simulink library "mjLib"  (R2025b)
settings: Solver=VariableStepAuto  StartTime=0.0  StopTime=10.0  RelTol=1e-3
settings Model: Creator=vmano  LastModifiedBy=Junch
settings OptimizationCC: ReuseModelBlockBuffer=off
settings DebuggingCC: UnconnectedInputMsg=warning  UnconnectedOutputMsg=warning  UnconnectedLineMsg=warning
settings ModelReferenceCC: EnableRefExpFcnMdlSchedulingChecks=on
settings RTWCC: GPUComputeCapability=3.5  DLArmComputeVersion=19.05

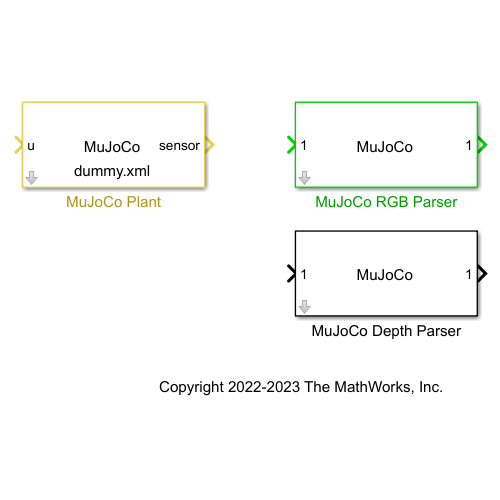
[thumbnail: Simulink's stored preview of the top-level diagram]
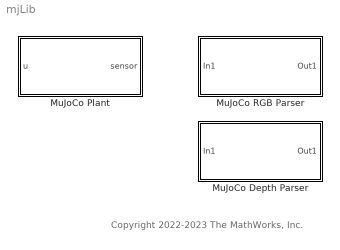
== system mjLib ==
  note: Copyright 2022-2023 The MathWorks, Inc.
  MuJoCo Depth Parser : Subsystem  mask{inputBusType=mj_bus_rgb_6338524502533525485, selectedCamera=camera, imageRows=480, imageCols=640, startingIndex=1, endingIndex=307200}
      mask prompts: inputBusType "Input Type"; selectedCamera "Select Camera"
      mask TypeOptions inputBusType: mj_bus_rgb_6338524502533525485
      mask Callback inputBusType:
      | inputBusType = get_param(gcb, 'inputBusType');
      | 
      | inputStruct = Simulink.Bus.createMATLABStruct(inputBusType);
      | 
      | mo = Simulink.Mask.get(gcb);
      | mo.Parameters(2).TypeOptions = fieldnames(inputStruct);
      mask TypeOptions selectedCamera: camera
      mask Callback selectedCamera:
      | inputBusType = get_param(gcb, 'inputBusType');
      | selectedCamera = get_param(gcb, 'selectedCamera');
      | 
      | inputStruct = Simulink.Bus.createMATLABStruct(inputBusType);
      | imageSize = size(inputStruct.(selectedCamera));
      | 
      | imageRows = imageSize(1);
      | imageCols = imageSize(2);
      | 
      | set_param(gcb, 'imageRows', num2str(imageRows));
      | set_param(gcb, 'imageCols', num2str(imageCols));
      | 
      | fields = fieldnames(inputStruct);
      | [~, camIndex] = ismember(selectedCamera, fields);
      | 
      | startingIndex = 1;
      | for i=1:(camIndex-1)
      |     imageSize = size(inputStruct.(fields{i}));
      |     startingIndex = startingIndex + imageSize(1)*imageSize(2);
      | end
      | endingIndex = startingIndex+imageSize(1) * imageSize(2) - 1;
      | 
      | set_param(gcb, 'startingIndex', num2str(startingIndex));
      | set_param(gcb, 'endingIndex', num2str(endingIndex));
      mask DialogControl Control2 Prompt: Refresh
      mask DialogControl Control2 Callback:
      | mo = Simulink.Mask.get(gcb);
      | mo.Parameters(1).TypeOptions = evalin('base', "who('mj_bus_rgb*')");
      mask Display:
      | color('black')
      | text(0.5, 0.5, 'MuJoCo', 'horizontalAlignment', 'center')
  MuJoCo Plant : Subsystem  mask(MuJoCo Plant){controlBus=[], sensorBus=mj_bus_sensor_7979902499018342666, controlLength=[], sensorLength=[], rgbLength=[], depthLength=[], sampleTime=0.005, xmlFileRel=dummy.xml, xmlFile=D:\robotics\mujoco_blocks\dummy.xml, renderingType=Global, vsync=off, visualFPS=60, zoomLevel=1, windowWidth=800, windowHeight=800, showSiteTrajectory=off, trajectorySiteName=, znear=0.059256, zfar=296.2816, cameraOutputEnabled=off, cameraSampleTime=0.020, rgbOutOption=on, depthOutOption=off, controlInterfaceType=Vector}
      mask prompts: renderingType "Type"; visualFPS "FPS"; zoomLevel "Zoom"; windowWidth "Window width (px)"; windowHeight "Window height (px)"; showSiteTrajectory "Show Site Trajectory"; trajectorySiteName "Site Name"; cameraOutputEnabled "Camera Output"; cameraSampleTime "Sample Time"; rgbOutOption "RGB Output"; depthOutOption "Depth Output"; controlInterfaceType "Interface"
      mask help:
      | This block provides an interface to MuJoCo™ physics engine.
      | It sets control inputs, steps the engine and outputs sensor/camera.
      |
      | Inputs, sensors, cameras and sample time information is obtained from the model XML.
      |
      | Control inputs are provided either as a non-virtual bus or vector.
      | Sensors are output as a non-virtual bus.
      | Camera data is output as a vector which can be decoded using MuJoCo RGB/Depth Parser blocks.
      mask init:
      | [controlBus, sensorBus, rgbBus, depthBus, dataLengths] = mj_initbus(xmlFile, cameraOutputEnabled);
      |     controlLength = double(dataLengths(1));
      |     sensorLength = double(dataLengths(2));
      |     rgbLength = double(dataLengths(3));
      |     depthLength = double(dataLengths(4)) * double(depthOutOption);
      |     mj_maskinit;
      mask Callback xmlFileRel:
      | relpath = get_param(gcb, 'xmlFileRel');
      | 
      | abspath = which(relpath);
      | if isempty(abspath)
      |     abspath = relpath;
      | end
      | set_param(gcb, 'xmlFile', abspath);
      mask TypeOptions renderingType: Local | Global | None
      mask TypeOptions controlInterfaceType: Bus | Vector
      mask DialogControl Container3 Prompt: Model Info
      mask DialogControl controlBusText Prompt: Control Vector Type: [armMotor]
      mask DialogControl sensorBusText Prompt: Sensor Bus Type: mj_bus_sensor_15738467249377022003
      mask DialogControl rgbBusText Prompt: RGB Bus Type: NA
      mask DialogControl depthBusText Prompt: Depth Bus Type: NA
      mask DialogControl sampleTimeText Prompt: Sample Time: 0.005
      mask DialogControl Container10 Prompt: Model
      mask DialogControl getFileButton Prompt: Browse
      mask DialogControl getFileButton Callback:
      | oldPath = get_param(gcb, 'xmlFile');
      | [file, path] = uigetfile({'*.xml;*.urdf'}, 'File Selector', oldPath);
      | if file~=0
      |     xml = fullfile(path, file);
      |     set_param(gcb, 'xmlFileRel', xml);
      | end
      mask DialogControl testStandaloneButton Prompt: Test
      mask DialogControl testStandaloneButton Callback: disp('Not implemented yet. Call simulate.exe inside 3p/mujoco folder')
      mask DialogControl Container12 Prompt: Rendering
      mask DialogControl Control11 Prompt: Rendering thread is common to all MuJoCo blocks and is used for rendering visualizer window along with all cameras
      mask DialogControl Container9 Prompt: Visualizer
      mask DialogControl Control10 Prompt: Visualizer renders frames at specified FPS. Display buffer swap timing is controlled separately via vsync option.
      mask DialogControl renderingType Tooltip: Local rendering creates a unique window for each MuJoCo block. Global tries to merge different block visuals into one window. None disables visualization
      mask DialogControl Container11 Prompt: Options
      mask DialogControl vsync Tooltip: Vsync blocks rendering thread until the monitor is ready to show the next frame. This prevents screen tearing effect. Vsync can slow down everything including physics loop.
      mask DialogControl visualFPS Tooltip: If Vsync is disabled, specify the FPS to show visuals at.
      mask DialogControl windowWidth Tooltip: Initial width of the visualization window. For Global rendering, the block that creates the shared window sets its size.
      mask DialogControl windowHeight Tooltip: Initial height of the visualization window. For Global rendering, the block that creates the shared window sets its size.
      mask DialogControl showSiteTrajectory Tooltip: Draw the world-space path of the selected site in the Local or Global window.
      mask DialogControl trajectorySiteName Tooltip: Exact name of a site in the loaded MJCF model. Required when Show Site Trajectory is selected.
      mask DialogControl Container13 Prompt: Camera
      mask DialogControl Control9 Prompt: Camera rendering runs in lockstep with physics engine.
      mask DialogControl cameraOutputEnabled Tooltip: Enable offscreen camera rendering and RGB/depth output ports.
      mask DialogControl depthOutOption Tooltip: Disable depth buffer processing to improve simulation speed.
      mask DialogControl Container7 Prompt: Control Inputs
      mask Display:
      | color('black')
      | text(0.5, 0.5, 'MuJoCo', 'horizontalAlignment', 'center')
      | [~, nameText, ext] = fileparts(get_param(gcb, 'xmlFile'));
      | text(0.5, 0.2, [nameText, ext], 'horizontalAlignment', 'center')
  MuJoCo RGB Parser : Subsystem  mask{inputBusType=mj_bus_rgb_6338524502533525485, selectedCamera=camera, imageRows=480, imageCols=640, startingIndex=1, endingIndex=921600}
      mask prompts: inputBusType "Input Type"; selectedCamera "Select Camera"
      mask TypeOptions inputBusType: mj_bus_rgb_4478678753310125630 | mj_bus_rgb_4479672711821839149
      mask Callback inputBusType:
      | inputBusType = get_param(gcb, 'inputBusType');
      | 
      | inputStruct = Simulink.Bus.createMATLABStruct(inputBusType);
      | 
      | mo = Simulink.Mask.get(gcb);
      | mo.Parameters(2).TypeOptions = fieldnames(inputStruct);
      mask TypeOptions selectedCamera: camera
      mask Callback selectedCamera:
      | inputBusType = get_param(gcb, 'inputBusType');
      | selectedCamera = get_param(gcb, 'selectedCamera');
      | 
      | inputStruct = Simulink.Bus.createMATLABStruct(inputBusType);
      | imageSize = size(inputStruct.(selectedCamera));
      | 
      | imageRows = imageSize(1);
      | imageCols = imageSize(2);
      | 
      | set_param(gcb, 'imageRows', num2str(imageRows));
      | set_param(gcb, 'imageCols', num2str(imageCols));
      | 
      | fields = fieldnames(inputStruct);
      | [~, camIndex] = ismember(selectedCamera, fields);
      | 
      | startingIndex = 1;
      | for i=1:(camIndex-1)
      |     imageSize = size(inputStruct.(fields{i}));
      |     startingIndex = startingIndex + imageSize(1)*imageSize(2)*imageSize(3);
      | end
      | endingIndex = startingIndex+imageSize(1) * imageSize(2)*imageSize(3) - 1;
      | 
      | set_param(gcb, 'startingIndex', num2str(startingIndex));
      | set_param(gcb, 'endingIndex', num2str(endingIndex));
      mask DialogControl Control2 Prompt: Refresh
      mask DialogControl Control2 Callback:
      | mo = Simulink.Mask.get(gcb);
      | mo.Parameters(1).TypeOptions = evalin('base', "who('mj_bus_rgb*')");
      mask Display:
      | color('black')
      | text(0.5, 0.5, 'MuJoCo', 'horizontalAlignment', 'center')

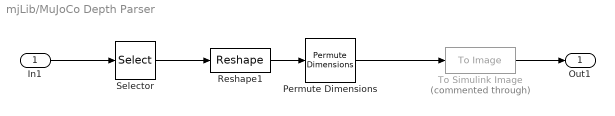
== system mjLib/MuJoCo Depth Parser ==
  In1 : Inport
  Permute Dimensions : PermuteDimensions  Order=[3 2 1]
  Reshape1 : Reshape  OutputDimensionality=Customize  OutputDimensions=[1,imageCols, imageRows]
  Selector : Selector  IndexOptions=Index vector (dialog)  Indices=startingIndex:endingIndex  OutputSizes=1
  To Simulink Image : ToImage  Commented=through  OutDataTypeStr=Simulink.ImageType(imageRows,imageCols,1,'ColorFormat','Grayscale','Layout','ColumnMajor','ClassUnderlying','single')
  Out1 : Outport
  wires:
  Reshape1/1 -> Permute Dimensions/1
  In1/1 -> Selector/1
  Selector/1 -> Reshape1/1
  To Simulink Image/1 -> Out1/1
  Permute Dimensions/1 -> To Simulink Image/1

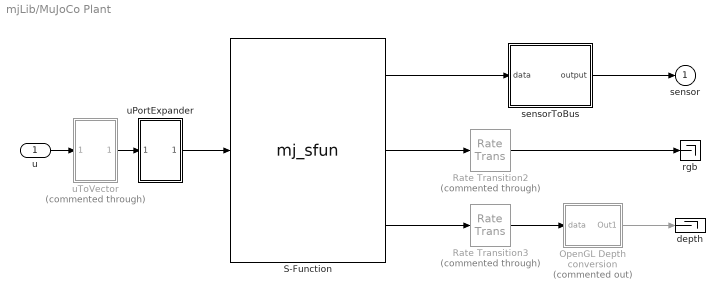
== system mjLib/MuJoCo Plant ==
  u : Inport  PortDimensions="[1  1]"
  OpenGL Depth conversion : Subsystem  Commented=on
  Rate Transition2 : RateTransition  Commented=through  OutPortSampleTime=cameraSampleTime
  Rate Transition3 : RateTransition  Commented=through  OutPortSampleTime=cameraSampleTime
  S-Function : S-Function  FunctionName=mj_sfun  Parameters=xmlFile, renderingType, controlLength, sensorLength, rgbLength, depthLength, vsync, visualFPS, cameraSampleTime, sampleTime, zoomLevel, windowWidth, windowHeight, depthOutOption, showSiteTrajectory, trajectorySiteName, cameraOutputEnabled  SFunctionDeploymentMode=off  EnableBusSupport=off
  depth : Terminator
  rgb : Terminator
  sensorToBus : Subsystem
  uPortExpander : Subsystem
  uToVector : Subsystem  Commented=through
  sensor : Outport
  wires:
  OpenGL Depth conversion/1(Out1) -> depth/1
  Rate Transition3/1 -> OpenGL Depth conversion/1(data)
  Rate Transition2/1 -> rgb/1
  S-Function/3 -> Rate Transition3/1
  S-Function/2 -> Rate Transition2/1
  uPortExpander/1(Out1) -> S-Function/1
  sensorToBus/1(output) -> sensor/1
  S-Function/1 -> sensorToBus/1(data)
  uToVector/1(Out1) -> uPortExpander/1(In1)
  u/1 -> uToVector/1(In1)

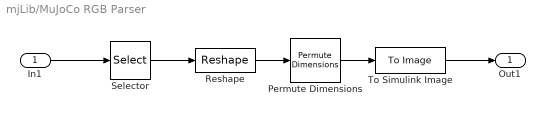
== system mjLib/MuJoCo RGB Parser ==
  In1 : Inport  OutDataTypeStr=uint8
  Permute Dimensions : PermuteDimensions  Order=[3 2 1]
  Reshape : Reshape  OutputDimensionality=Customize  OutputDimensions=[3,imageCols, imageRows]
  Selector : Selector  IndexOptions=Index vector (dialog)  Indices=startingIndex:endingIndex  OutputSizes=1
  To Simulink Image : ToImage  OutDataTypeStr=Simulink.ImageType(imageRows,imageCols,3)
  Out1 : Outport
  wires:
  Permute Dimensions/1 -> To Simulink Image/1
  In1/1 -> Selector/1
  Reshape/1 -> Permute Dimensions/1
  To Simulink Image/1 -> Out1/1
  Selector/1 -> Reshape/1

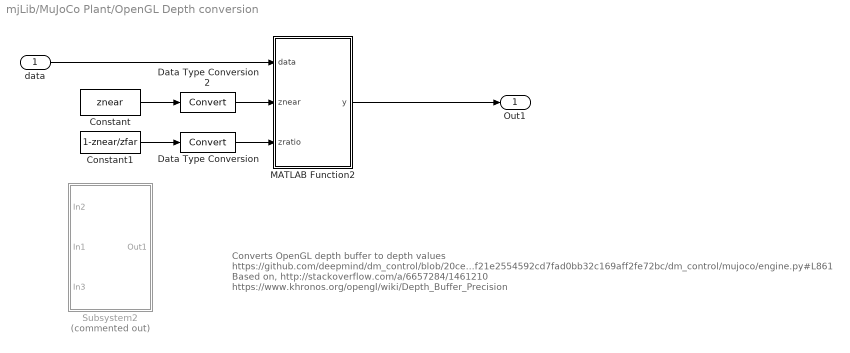
== system mjLib/MuJoCo Plant/OpenGL Depth conversion ==
  note: Converts OpenGL depth buffer to depth values
      | https://github.com/deepmind/dm_control/blob/20cef21e2554592cd7fad0bb32c169aff2fe72bc/dm_control/mujoco/engine.py#L861
      | Based on,
      | http://stackoverflow.com/a/6657284/1461210
      | https://www.khronos.org/opengl/wiki/Depth_Buffer_Precision
  data : Inport
  Constant : Constant  Value=znear
  Constant1 : Constant  Value=1-znear/zfar
  Data Type Conversion : DataTypeConversion  SaturateOnIntegerOverflow=off  RndMeth=Floor
  Data Type Conversion2 : DataTypeConversion  SaturateOnIntegerOverflow=off  RndMeth=Floor
  MATLAB Function2 : MATLAB Function  TreatAsAtomicUnit=on
  Subsystem2 : Subsystem  Commented=on
  Out1 : Outport
  wires:
  MATLAB Function2/1(y) -> Out1/1
  Data Type Conversion/1 -> MATLAB Function2/3(zratio)
  data/1 -> MATLAB Function2/1(data)
  Data Type Conversion2/1 -> MATLAB Function2/2(znear)
  Constant1/1 -> Data Type Conversion/1
  Constant/1 -> Data Type Conversion2/1

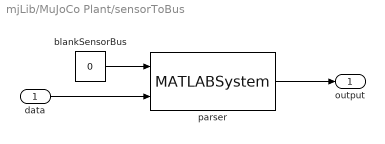
== system mjLib/MuJoCo Plant/sensorToBus ==
  data : Inport
  blankSensorBus : Constant  Value=0  OutDataTypeStr=Bus: mj_bus_sensor_15738467249377022003
  parser : MATLABSystem  System=mj_sensor_parser  OutputBusName=mj_bus_sensor_15738467249377022003  SimulateUsing=Code generation
      mask Type: mj_sensor_parser
  output : Outport
  wires:
  parser/1 -> output/1
  data/1 -> parser/2
  blankSensorBus/1 -> parser/1

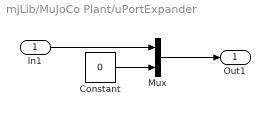
== system mjLib/MuJoCo Plant/uPortExpander ==
  In1 : Inport
  Constant : Constant  Value=0
  Mux : Mux  Inputs=2
  Out1 : Outport
  wires:
  Constant/1 -> Mux/2
  Mux/1 -> Out1/1
  In1/1 -> Mux/1

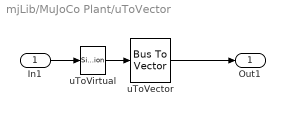
== system mjLib/MuJoCo Plant/uToVector ==
  In1 : Inport
  uToVector : BusToVector
  uToVirtual : SignalConversion  ConversionOutput=Virtual bus  OverrideOpt=off
  Out1 : Outport
  wires:
  uToVector/1 -> Out1/1
  In1/1 -> uToVirtual/1
  uToVirtual/1 -> uToVector/1

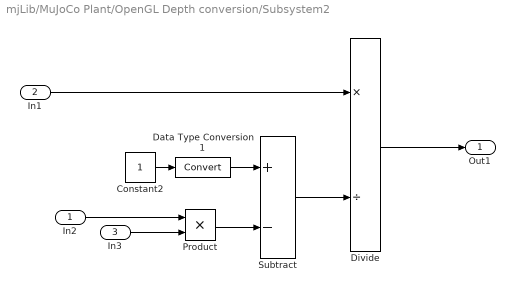
== system mjLib/MuJoCo Plant/OpenGL Depth conversion/Subsystem2 ==
  In2 : Inport
  In1 : Inport  Port=2
  In3 : Inport  Port=3
  Constant2 : Constant
  Data Type Conversion1 : DataTypeConversion  SaturateOnIntegerOverflow=off  RndMeth=Floor
  Divide : Product  Inputs=*/
  Product : Product
  Subtract : Sum  Inputs=+-
  Out1 : Outport
  wires:
  In3/1 -> Product/2
  Subtract/1 -> Divide/2
  In1/1 -> Divide/1
  Divide/1 -> Out1/1
  Constant2/1 -> Data Type Conversion1/1
  Product/1 -> Subtract/2
  In2/1 -> Product/1
  Data Type Conversion1/1 -> Subtract/1

== matlab function mjLib/MuJoCo Plant/OpenGL Depth conversion/MATLAB Function2 ==
  data: data input; znear input; zratio input; y output
function y = fcn(data, znear, zratio)
y = znear./(1-data*zratio);
